simulink model "matthew"  (R2026a)
settings: Solver=FixedStepAuto  StopTime=10
values from neighbouring files (symbols this model uses):
  Kd = 40.0 / 400.0    (= 0.1)    [matthew_ZOH.m]
  Ki = (2*final_Kloop - 2*Kp) / T    (= 77.57225)    [matthew_ZOH.m]
  Kp = (final_Kloop + final_Kloop * final_czero) / 2    (= 1.594313875)    [matthew_ZOH.m]
  T = sisoinit(4)    [matthew_ZOH.m]    (also in plant_ZOH.m)
libraries: cstblocks_lti x3
settings Model: Creator=ms110  LastModifiedBy=ms110

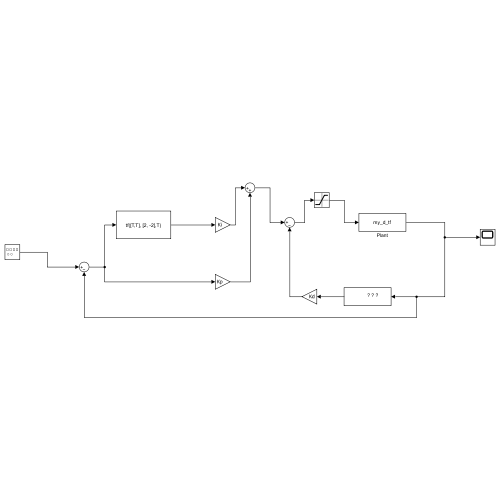
[thumbnail: Simulink's stored preview of the top-level diagram]
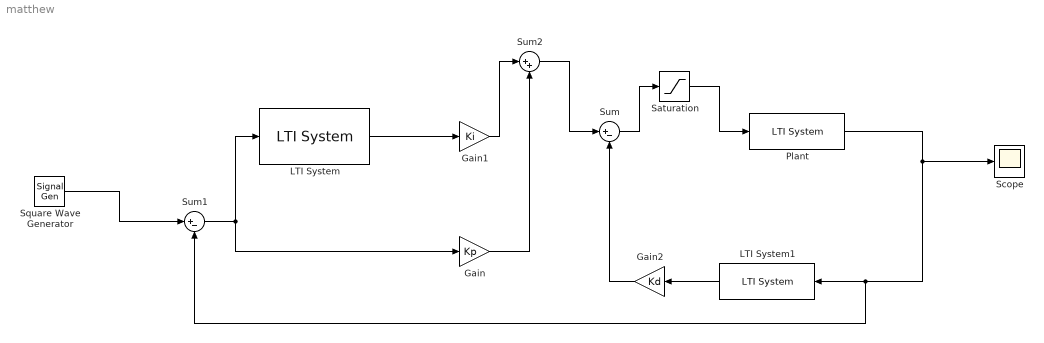
== system matthew ==
  Gain : Gain  Gain=Kp
  Gain1 : Gain  Gain=Ki
  Gain2 : Gain  Gain=Kd
  LTI System : cstblocks_lti/LTI System  sys=tf([T,T], [2, -2],T)  IC=[]  PadeOrder=0
      settings: LibrarySourceBlock=cstblocks/LTI System
  LTI System1 : cstblocks_lti/LTI System  sys="c2d(tf([500 0], [1 500]), T, \"tustin\")"  IC=[]  PadeOrder=0
      settings: LibrarySourceBlock=cstblocks/LTI System
  Plant : cstblocks_lti/LTI System  sys=my_d_tf  IC=[]  PadeOrder=0
      settings: LibrarySourceBlock=cstblocks/LTI System
  Saturation : Saturate  UpperLimit=10  LowerLimit=-10
  Scope : Scope
      settings: ActiveDisplayYMinimum=-1.6619879571267457  ActiveDisplayYMaximum=1.2590201853569494
  Square Wave Generator : SignalGenerator  WaveForm=square  Frequency=.25
  Sum : Sum  Inputs=|+-
  Sum1 : Sum  Inputs=|+-
  Sum2 : Sum  Inputs=|++
  wires:
  Plant/1 -> Sum1/2, LTI System1/1, Scope/1
  LTI System1/1 -> Gain2/1
  Gain2/1 -> Sum/2
  Sum1/1 -> Gain/1, LTI System/1
  LTI System/1 -> Gain1/1
  Gain1/1 -> Sum2/1
  Gain/1 -> Sum2/2
  Sum2/1 -> Sum/1
  Square Wave Generator/1 -> Sum1/1
  Sum/1 -> Saturation/1
  Saturation/1 -> Plant/1
